simulink model "Q1"  (R2025b)
settings: Solver=VariableStepAuto  StartTime=0.0  StopTime=10.0  MaxStep=1e-3  RelTol=1e-3
settings Model: Creator=dkaze  LastModifiedBy=dkaze

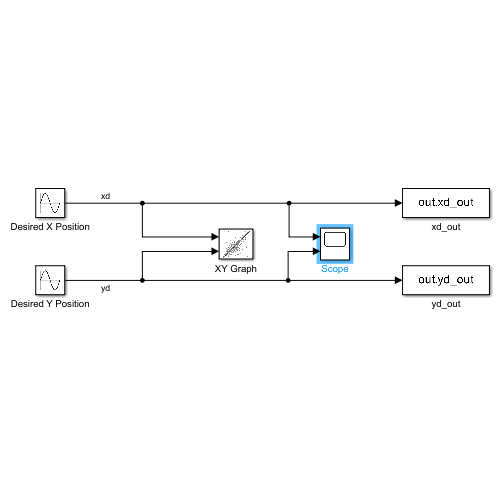
[thumbnail: Simulink's stored preview of the top-level diagram]
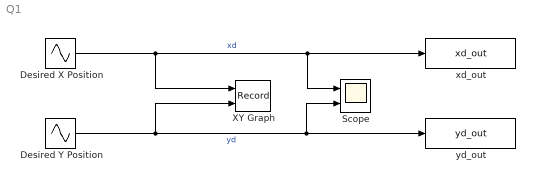
== system Q1 ==
  Desired X Position : Sin  Amplitude=10  Bias=50  Frequency=2*pi/5  Phase=pi/2  SampleTime=0
  Desired Y Position : Sin  Amplitude=10  Bias=20  Frequency=2*pi/5  SampleTime=0
  Scope : Scope  NumInputPorts=2
      settings: Title=Desired Cartesian Position Trajectories  ActiveDisplayYMinimum=3.7500000000000018  ActiveDisplayYMaximum=66.25  YLabel=Position (cm)
  XY Graph : Record  NumPorts=2.0  FileSettingsInternal="{\"entries\":[{\"content\":{\"excelSettings\":{\"content\":{},\"type\":\"Streamout.ExcelSettings\"},\"parquetSettings\":{\"content\":{},\"type\":\"Streamout.ParquetSettings\"}},\"type\":\"Streamout.FileSettingStorage\",\"uuid\":\"\"}],\"packageUris\":[\"http:\\/\\/schema.mathworks.com\\/mf0\\/streamout_blocks\\/R2020a\"],\"version\":\"1.0\"}"  FrameSettings=[0, 0]  Layout=[1 1]  SignalsInternal="{\"entries\":[{\"content\":{\"signals\":[{\"content\":{\"blockPath\":[],\"dimensions\":[1],\"domain\":\"\",\"lineColor\":\"#a2142f\",\"plots\":[ 1 ],\"port\":1,\"signalID\":1,\"signalName\":\"xd\"},\"type\":\"RecordBlkView.Signal\",\"uuid\":\"\"},{\"content\":{\"blockPath\":[],\"dimensions\":[1],\"domain\":\"\",\"lineColor\":\"#139fff\",\"plots\":[ 1 ],\"port\":2,\"signalID\":2,\"signalName\":\"yd\"},\"type\":\"RecordBlkView.Signal\",\"uuid\":\"\"}]},\"type\":\"RecordBlkView.InputSignals\",\"uuid\":\"\"}],\"packageUris\":[\"http:\\/\\/schema.mathworks.com\\/mf0\\/streamout_blocks\\/R2020a\"],\"version\":\"1.0\"}"  VisualizationBindings="{\"xyplotplugin\":{\"info\":[{\"series\":[{\"bindingParametersList\":[{\"parameter\":\"X-Axis\",\"signalID\":1,\"signalName\":\"xd\"},{\"parameter\":\"Y-Axis\",\"signalID\":2,\"signalName\":\"yd\"}],\"seriesID\":0}],\"subplotID\":1}]}}"  CompatibilityTag=XY
  xd_out : ToWorkspace  VariableName=xd_out  SaveFormat=Timeseries  SampleTime=-1
  yd_out : ToWorkspace  VariableName=yd_out  SaveFormat=Timeseries  SampleTime=-1
  wires:
  Desired X Position/1 -> XY Graph/1, Scope/1, xd_out/1  "xd"
  Desired Y Position/1 -> XY Graph/2, Scope/2, yd_out/1  "yd"
